simulink model "x3D_FSC_integrale"  (R2024b)
settings: Solver=FixedStepAuto  StartTime=0.0  StopTime=inf  FixedStep=0.001  RelTol=1e-3  EnableMultiTasking=on
undefined symbols (not defined in the file or in its folder): DiscIntNeverNeededParam
libraries: px4Sensorslib x5, matrix_library x4, px4Peripheralslib x1, cstblocks x1
settings Model: SimulationMode=external  ExtModeTrigDuration=10  Creator=ArriGE66  LastModifiedBy=xippa
settings SolverCC: PositivePriorityOrder=on
settings OptimizationCC: EnhancedBackFolding=on  PassReuseOutputArgsAs=Individual arguments  ZeroExternalMemoryAtStartup=off  ZeroInternalMemoryAtStartup=off  MaxStackSize=64  OptimizeBlockOrder=speed  DifferentSizesBufferReuse=on  OptimizationCustomize=off  EfficientTunableParamExpr=on
settings DebuggingCC: ParameterTunabilityLossMsg=error
settings HardwareCC: ProdBitPerPointer=32  ProdBitPerSizeT=32  ProdBitPerPtrDiffT=32  ProdLargestAtomicInteger=Long  ProdLargestAtomicFloat=Double  ProdWordSize=32  ProdLongLongMode=on  ProdHWDeviceType=ARM Compatible->ARM Cortex
settings SFSimCC: MATLABDynamicMemAlloc=off  SimTargetLang=C++
settings RTWCC: Description=Embedded Coder  SystemTargetFile=ert.tlc  HardwareBoard=PX4 Cube Orange  TemplateMakefile=ert_default_tmf  Toolchain=GNU Tools for PX4 Autopilots  TargetLang=C++  GPUComputeCapability=3.5
settings CodeAppCC: ForceParamTrailComments=on  IgnoreCustomStorageClasses=off  OperatorAnnotations=on  SimulinkDataObjDesc=on  SFDataObjDesc=on  InsertBlockDesc=on
settings ERTTargetCC: SupportVariableSizeSignals=on  ExtMode=on  ExtModeTransport=3  ExtModeStaticAlloc=on  ExtModeStaticAllocSize=1024  ExtModeMexFile=ext_xcp  ExtModeMexArgs=1 COM10 3000000  ExtModeIntrfLevel=Level2 - Open  InlinedParameterPlacement=Hierarchical  DynamicArrayContainerType=coder::array

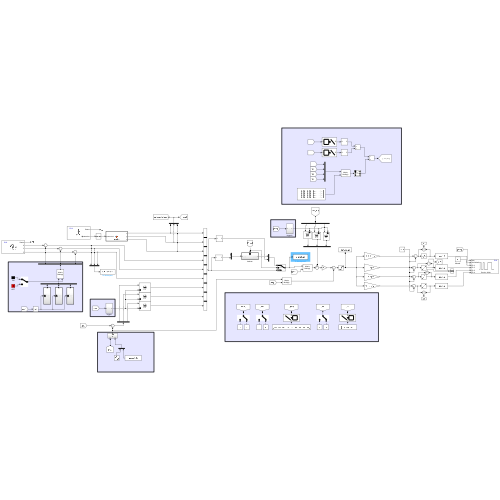
[thumbnail: Simulink's stored preview of the top-level diagram]
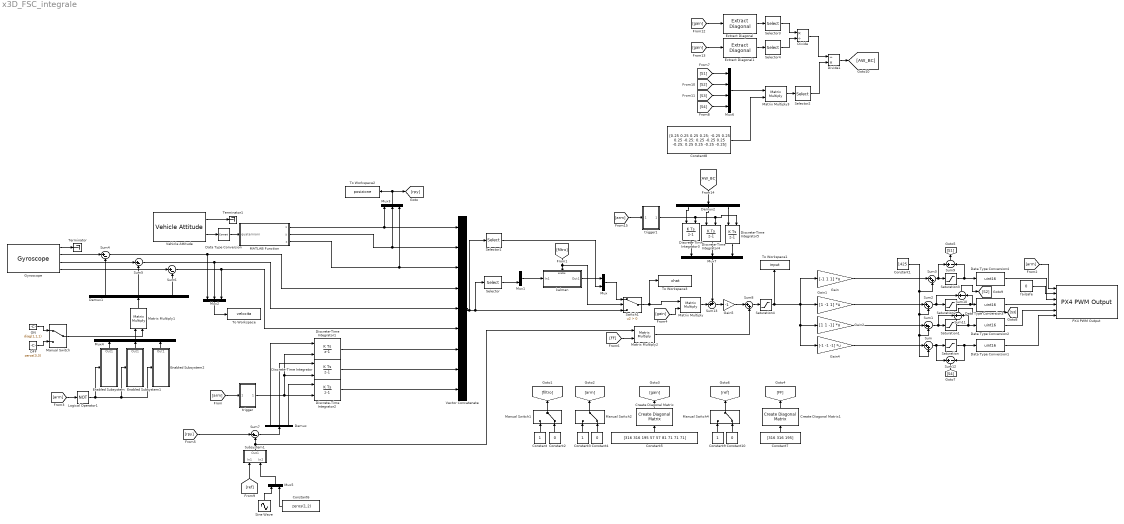
== system x3D_FSC_integrale ==
  Constant : Constant
  Constant1 : Constant  Value=1425  SampleTime=0.01
  Constant10 : Constant  Value=0
  Constant2 : Constant  Value=0
  Constant3 : Constant
  Constant4 : Constant  Value=0
  Constant5 : Constant  Value=[316 316 195 57 57 81 71 71 71]
  Constant6 : Constant  Value=zeros(1,2)
  Constant7 : Constant  Value=[316 316 195]
  Constant8 : Constant  Value=|
      | [0.25	0.25	0.25	0.25;
      | -0.25	0.25	0.25	-0.25;
      | 0.25	-0.25	0.25	-0.25;
      | 0.25	0.25	-0.25	-0.25]
  Constant9 : Constant
  Create Diagonal Matrix : matrix_library/Create Diagonal Matrix
      settings: LibrarySourceBlock=|
      | simulink/Matrix
      | Operations/Create Diagonal
      | Matrix
  Create Diagonal Matrix1 : matrix_library/Create Diagonal Matrix
      settings: LibrarySourceBlock=|
      | simulink/Matrix
      | Operations/Create Diagonal
      | Matrix
  Data Type Conversion : DataTypeConversion  SaturateOnIntegerOverflow=off  RndMeth=Floor
  Data Type Conversion{1..4} (4 alike) : DataTypeConversion  OutDataTypeStr=uint16  SaturateOnIntegerOverflow=off  RndMeth=Floor
  Demux : Demux  Outputs=3
  Demux1 : Demux  Outputs=3
  Demux2 : Demux  Outputs=3
  Discrete-Time Integrator{,1..5} (6 alike) : DiscreteIntegrator  ExternalReset=level  SampleTime=-1  ICPrevOutput=DiscIntNeverNeededParam  ICPrevScaledInput=DiscIntNeverNeededParam
  Divide : Product  Inputs=*/
  Divide1 : Product  Inputs=/*
  Enabled Subsystem : Subsystem  TreatAsAtomicUnit=on
  Enabled Subsystem1 : Subsystem  TreatAsAtomicUnit=on
  Enabled Subsystem2 : Subsystem  TreatAsAtomicUnit=on
  Extract Diagonal : matrix_library/Extract Diagonal
      settings: LibrarySourceBlock=|
      | simulink/Matrix
      | Operations/Extract Diagonal
  Extract Diagonal1 : matrix_library/Extract Diagonal
      settings: LibrarySourceBlock=|
      | simulink/Matrix
      | Operations/Extract Diagonal
  Gain : Gain  Gain=[-1 1 1]  Multiplication=Matrix(K*u)
  Gain1 : Gain  Gain=[1 -1 1]  Multiplication=Matrix(K*u)
  Gain2 : Gain  Gain=[1 1 -1]  Multiplication=Matrix(K*u)
  Gain4 : Gain  Gain=[-1 -1 -1]  Multiplication=Matrix(K*u)
  Gain5 : Gain  Gain=-1
  Gyroscope : px4Sensorslib/Gyroscope  uorbTimeStamp=off  BlockingMode=off  BlockTimeout=1e-3  sampleTime=0.01
  Logical Operator1 : Logic  Operator=NOT  AllPortsSameDT=off  OutDataTypeStr=boolean
  MATLAB Function : MATLAB Function  TreatAsAtomicUnit=on
  Manual Switch : ManualSwitch
  Manual Switch1 : ManualSwitch  CurrentSetting=0
  Manual Switch2 : ManualSwitch  CurrentSetting=0
  Manual Switch4 : ManualSwitch  CurrentSetting=0
  Matrix Multiply{,1..3} (4 alike) : Product  Multiplication=Matrix(*)
  Mux : Mux  Inputs=2
  Mux1 : Mux  Inputs=2
  Mux{2..4,7} (4 alike) : Mux  Inputs=3
  Mux5 : Mux  Inputs=2
  Mux6 : Mux
  OFF : Constant  Value=zeros(3,3)
  ON : Constant  Value=diag(1,1,1)
  PX4 PWM Output : px4Peripheralslib/PX4 PWM Output  pwmDevice=Main  pwmChannel1_=on  pwmChannel2_=on  pwmChannel3_=on  pwmChannel4_=on  pwmChannel5_=off  pwmChannel6_=off  pwmChannel7_=off  pwmChannel8_=off
  Saturation{,1..3} (4 alike) : Saturate  UpperLimit=1750  LowerLimit=1050
  Saturation4 : Saturate
  Selector : Selector  InputPortWidth=9  IndexOptions=Index vector (dialog)  Indices=[1:6]  OutputSizes=1
  Selector1 : Selector  InputPortWidth=9  IndexOptions=Index vector (dialog)  Indices=[7 8 9]  OutputSizes=1
  Selector2 : Selector  InputPortWidth=4  IndexOptions=Index vector (dialog)  Indices=[2:4]  OutputSizes=1
  Selector3 : Selector  InputPortWidth=9  IndexOptions=Index vector (dialog)  Indices=[1 2 3]  OutputSizes=1
  Selector4 : Selector  InputPortWidth=9  IndexOptions=Index vector (dialog)  Indices=[7 8 9]  OutputSizes=1
  Sine Wave : Sin  Amplitude=0.1  SampleTime=0.01
  Subsystem1 : Subsystem
  Sum{,1..3,8} (5 alike) : Sum  Inputs=|++
  Sum{9..12} (4 alike) : Sum  Inputs=+|-
  Sum13 : Sum  Inputs=++|
  Sum{4..7} (4 alike) : Sum  Inputs=|+-
  Switch1 : Switch  Criteria=u2 > Threshold  SaturateOnIntegerOverflow=off  InputSameDT=off
  Terminator : Terminator
  Terminator1 : Terminator
  To Workspace : ToWorkspace  VariableName=velocita  SaveFormat=Timeseries  SampleTime=-1
  To Workspace1 : ToWorkspace  VariableName=input  SaveFormat=Timeseries  SampleTime=-1
  To Workspace2 : ToWorkspace  VariableName=posizione  SaveFormat=Timeseries  SampleTime=-1
  To Workspace3 : ToWorkspace  VariableName=xhat  SaveFormat=Timeseries  SampleTime=-1
  Vector Concatenate : Concatenate  NumInputs=9
  Vehicle Attitude : px4Sensorslib/Vehicle Attitude  rollRate=off  pitchRate=off  yawRate=off  quaternion=on  uorbTimeStamp=off  BlockingMode=off  BlockTimeout=0.001  sampleTime=0.01
  failsafe : Constant  Value=0  OutDataTypeStr=boolean  SampleTime=0.01
  kalman : Subsystem  TreatAsAtomicUnit=on
  trigger : Subsystem
  trigger1 : Subsystem
  wires:
  Data Type Conversion2/1 -> PX4 PWM Output/5
  Data Type Conversion1/1 -> PX4 PWM Output/6
  failsafe/1 -> PX4 PWM Output/2
  Vehicle Attitude/2 -> Data Type Conversion/1
  Vehicle Attitude/1 -> Terminator1/1
  Data Type Conversion3/1 -> PX4 PWM Output/4
  Gain/1 -> Sum3/1
  Saturation3/1 -> Sum9/2, Data Type Conversion4/1
  Data Type Conversion4/1 -> PX4 PWM Output/3
  Sum3/1 -> Sum9/1, Saturation3/1
  Constant1/1 -> Sum/2, Sum1/2, Sum2/2, Sum3/2
  Vector Concatenate/1 -> Selector1/1, Selector/1, Switch1/3
  Gain1/1 -> Sum2/1
  Gain2/1 -> Sum1/1
  Gain4/1 -> Sum/1
  Selector/1 -> Mux1/2
  [filtro] -> Switch1/2, kalman/Enable
  kalman/1(Out1) -> Mux/1
  Selector1/1 -> Mux/2
  Mux/1 -> Switch1/1
  Mux1/1 -> kalman/1(In1)
  Data Type Conversion/1 -> MATLAB Function/1(quaternioni)
  Switch1/1 -> To Workspace3/1, Matrix Multiply/1
  trigger/1(Out1) -> Discrete-Time Integrator1/2, Discrete-Time Integrator/2, Discrete-Time Integrator2/2
  [arm] -> trigger/1(In1)
  Sum4/1 -> Vector Concatenate/4, Mux2/1
  ON/1 -> Manual Switch/1
  Gyroscope/4 -> Sum6/1
  Manual Switch/1 -> Matrix Multiply1/2
  Demux1/2 -> Sum5/2
  Matrix Multiply1/1 -> Demux1/1
  Gyroscope/2 -> Sum4/1
  Gyroscope/3 -> Sum5/1
  OFF/1 -> Manual Switch/2
  Sum5/1 -> Vector Concatenate/5, Mux2/2
  Demux1/3 -> Sum6/2
  Demux1/1 -> Sum4/2
  Gyroscope/1 -> Terminator/1
  Sum6/1 -> Mux2/3, Vector Concatenate/6
  Logical Operator1/1 -> Enabled Subsystem2/Enable, Enabled Subsystem1/Enable, Enabled Subsystem/Enable
  Enabled Subsystem2/1(Out1) -> Mux4/3
  Enabled Subsystem/1(Out1) -> Mux4/1
  [arm] -> Logical Operator1/1
  Enabled Subsystem1/1(Out1) -> Mux4/2
  Mux4/1 -> Matrix Multiply1/1
  Manual Switch1/1 -> [filtro]
  Constant2/1 -> Manual Switch1/2
  Constant/1 -> Manual Switch1/1
  [arm] -> PX4 PWM Output/1
  Constant3/1 -> Manual Switch2/1
  Manual Switch2/1 -> [arm]
  Constant4/1 -> Manual Switch2/2
  [gain] -> Matrix Multiply/2
  Create Diagonal Matrix/1 -> [gain]
  Constant5/1 -> Create Diagonal Matrix/1
  Mux2/1 -> To Workspace/1
  MATLAB Function/1(x) -> Mux3/1, Vector Concatenate/1
  MATLAB Function/2(y) -> Mux3/2, Vector Concatenate/2
  MATLAB Function/3(z) -> Mux3/3, Vector Concatenate/3
  Discrete-Time Integrator1/1 -> Vector Concatenate/7
  Discrete-Time Integrator/1 -> Vector Concatenate/8
  Discrete-Time Integrator2/1 -> Vector Concatenate/9
  Mux3/1 -> [rpy], To Workspace2/1
  Manual Switch4/1 -> [ref]
  Constant9/1 -> Manual Switch4/1
  Constant10/1 -> Manual Switch4/2
  [ref] -> Subsystem1/1(In1)
  Sine Wave/1 -> Mux5/1
  Mux5/1 -> Subsystem1/2(In2)
  Constant6/1 -> Mux5/2
  [rpy] -> Sum7/1
  Sum7/1 -> Demux/1
  Demux/1 -> Discrete-Time Integrator1/1
  Demux/2 -> Discrete-Time Integrator/1
  Demux/3 -> Discrete-Time Integrator2/1
  Gain5/1 -> Sum8/1
  Sum8/1 -> Saturation4/1
  Matrix Multiply2/1 -> Sum8/2
  Subsystem1/1(Out1) -> Matrix Multiply2/1, Sum7/2
  [FF] -> Matrix Multiply2/2
  Create Diagonal Matrix1/1 -> [FF]
  Constant7/1 -> Create Diagonal Matrix1/1
  Saturation4/1 -> Gain4/1, Gain2/1, Gain1/1, Gain/1, To Workspace1/1
  Saturation2/1 -> Sum10/2, Data Type Conversion3/1
  Sum2/1 -> Sum10/1, Saturation2/1
  Saturation1/1 -> Sum11/2, Data Type Conversion2/1
  Sum1/1 -> Sum11/1, Saturation1/1
  Saturation/1 -> Sum12/2, Data Type Conversion1/1
  Sum/1 -> Sum12/1, Saturation/1
  Sum9/1 -> [S1]
  Sum12/1 -> [S4]
  Sum11/1 -> [S3]
  Sum10/1 -> [S2]
  [S2] -> Mux6/2
  [S1] -> Mux6/1
  [S3] -> Mux6/3
  [S4] -> Mux6/4
  Mux6/1 -> Matrix Multiply3/1
  Constant8/1 -> Matrix Multiply3/2
  Matrix Multiply3/1 -> Selector2/1
  [gain] -> Extract Diagonal/1
  Extract Diagonal/1 -> Selector3/1
  [gain] -> Extract Diagonal1/1
  Extract Diagonal1/1 -> Selector4/1
  Selector3/1 -> Divide/1
  Selector4/1 -> Divide/2
  Divide/1 -> Divide1/1
  Selector2/1 -> Divide1/2
  Divide1/1 -> [AW_BC]
  Matrix Multiply/1 -> Sum13/2
  [AW_BC] -> Demux2/1
  [arm] -> trigger1/1(In1)
  Demux2/3 -> Discrete-Time Integrator5/1
  Demux2/2 -> Discrete-Time Integrator4/1
  Demux2/1 -> Discrete-Time Integrator3/1
  trigger1/1(Out1) -> Discrete-Time Integrator5/2, Discrete-Time Integrator4/2, Discrete-Time Integrator3/2
  Sum13/1 -> Gain5/1
  Discrete-Time Integrator3/1 -> Mux7/1
  Discrete-Time Integrator5/1 -> Mux7/3
  Discrete-Time Integrator4/1 -> Mux7/2
  Mux7/1 -> Sum13/1

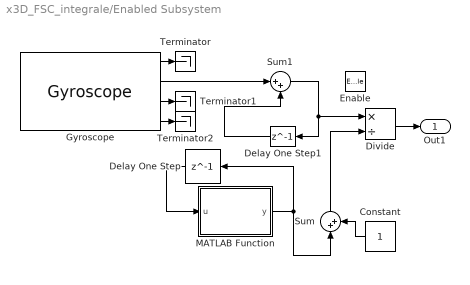
== system x3D_FSC_integrale/Enabled Subsystem ==
  Enable : EnablePort
  Constant : Constant
  Delay One Step : Delay  DelayLength=1
  Delay One Step1 : Delay  DelayLength=1
  Divide : Product  Inputs=*/
  Gyroscope : px4Sensorslib/Gyroscope  uorbTimeStamp=off  BlockingMode=off  BlockTimeout=1e-3  sampleTime=0.01
  MATLAB Function : MATLAB Function  TreatAsAtomicUnit=on
  Sum : Sum  Inputs=|++
  Sum1 : Sum  Inputs=|++
  Terminator : Terminator
  Terminator1 : Terminator
  Terminator2 : Terminator
  Out1 : Outport
  wires:
  Divide/1 -> Out1/1
  Sum1/1 -> Delay One Step1/1, Divide/1
  Sum/1 -> Divide/2
  Constant/1 -> Sum/2
  MATLAB Function/1(y) -> Delay One Step/1, Sum/1
  Delay One Step/1 -> MATLAB Function/1(u)
  Delay One Step1/1 -> Sum1/2
  Gyroscope/4 -> Terminator2/1
  Gyroscope/3 -> Terminator1/1
  Gyroscope/1 -> Terminator/1
  Gyroscope/2 -> Sum1/1

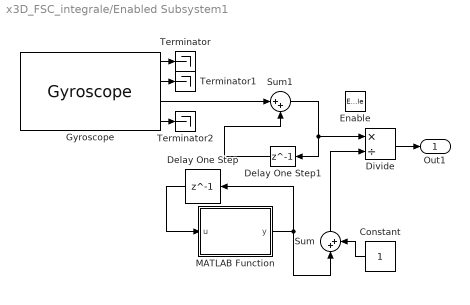
== system x3D_FSC_integrale/Enabled Subsystem1 ==
  Enable : EnablePort
  Constant : Constant
  Delay One Step : Delay  DelayLength=1
  Delay One Step1 : Delay  DelayLength=1
  Divide : Product  Inputs=*/
  Gyroscope : px4Sensorslib/Gyroscope  uorbTimeStamp=off  BlockingMode=off  BlockTimeout=1e-3  sampleTime=0.01
  MATLAB Function : MATLAB Function  TreatAsAtomicUnit=on
  Sum : Sum  Inputs=|++
  Sum1 : Sum  Inputs=|++
  Terminator : Terminator
  Terminator1 : Terminator
  Terminator2 : Terminator
  Out1 : Outport
  wires:
  Divide/1 -> Out1/1
  Sum1/1 -> Delay One Step1/1, Divide/1
  Sum/1 -> Divide/2
  Constant/1 -> Sum/2
  MATLAB Function/1(y) -> Delay One Step/1, Sum/1
  Delay One Step/1 -> MATLAB Function/1(u)
  Delay One Step1/1 -> Sum1/2
  Gyroscope/4 -> Terminator2/1
  Gyroscope/1 -> Terminator/1
  Gyroscope/3 -> Sum1/1
  Gyroscope/2 -> Terminator1/1

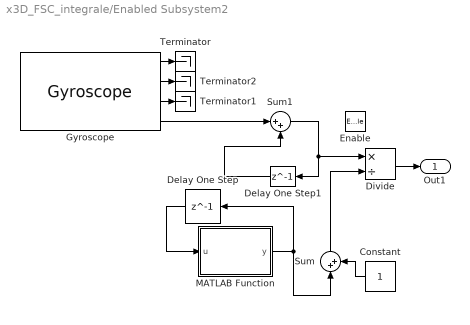
== system x3D_FSC_integrale/Enabled Subsystem2 ==
  Enable : EnablePort
  Constant : Constant
  Delay One Step : Delay  DelayLength=1
  Delay One Step1 : Delay  DelayLength=1
  Divide : Product  Inputs=*/
  Gyroscope : px4Sensorslib/Gyroscope  uorbTimeStamp=off  BlockingMode=off  BlockTimeout=1e-3  sampleTime=0.01
  MATLAB Function : MATLAB Function  TreatAsAtomicUnit=on
  Sum : Sum  Inputs=|++
  Sum1 : Sum  Inputs=|++
  Terminator : Terminator
  Terminator1 : Terminator
  Terminator2 : Terminator
  Out1 : Outport
  wires:
  Divide/1 -> Out1/1
  Sum1/1 -> Delay One Step1/1, Divide/1
  Sum/1 -> Divide/2
  Constant/1 -> Sum/2
  MATLAB Function/1(y) -> Delay One Step/1, Sum/1
  Delay One Step/1 -> MATLAB Function/1(u)
  Delay One Step1/1 -> Sum1/2
  Gyroscope/3 -> Terminator1/1
  Gyroscope/1 -> Terminator/1
  Gyroscope/4 -> Sum1/1
  Gyroscope/2 -> Terminator2/1

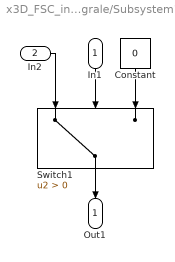
== system x3D_FSC_integrale/Subsystem1 ==
  In1 : Inport
  In2 : Inport  Port=2
  Constant : Constant  Value=0
  Switch1 : Switch  Criteria=u2 > Threshold  SaturateOnIntegerOverflow=off  InputSameDT=off
  Out1 : Outport
  wires:
  Switch1/1 -> Out1/1
  In1/1 -> Switch1/2
  Constant/1 -> Switch1/3
  In2/1 -> Switch1/1

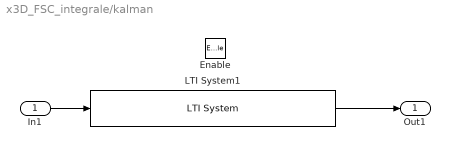
== system x3D_FSC_integrale/kalman ==
  In1 : Inport
  Enable : EnablePort
  LTI System1 : cstblocks/LTI System  sys=kalmand  IC=[0 0 0 0 0 0]  PadeOrder=0
  Out1 : Outport
  wires:
  In1/1 -> LTI System1/1
  LTI System1/1 -> Out1/1

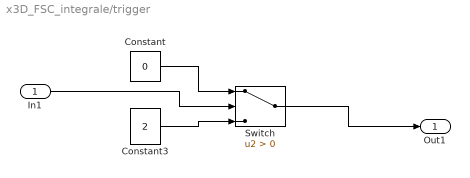
== system x3D_FSC_integrale/trigger ==
  In1 : Inport
  Constant : Constant  Value=0
  Constant3 : Constant  Value=2
  Switch : Switch  Criteria=u2 > Threshold  SaturateOnIntegerOverflow=off  InputSameDT=off
  Out1 : Outport
  wires:
  Constant/1 -> Switch/1
  Constant3/1 -> Switch/3
  Switch/1 -> Out1/1
  In1/1 -> Switch/2

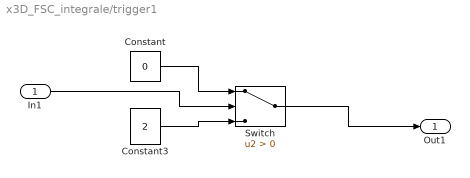
== system x3D_FSC_integrale/trigger1 ==
  In1 : Inport
  Constant : Constant  Value=0
  Constant3 : Constant  Value=2
  Switch : Switch  Criteria=u2 > Threshold  SaturateOnIntegerOverflow=off  InputSameDT=off
  Out1 : Outport
  wires:
  Constant/1 -> Switch/1
  Constant3/1 -> Switch/3
  Switch/1 -> Out1/1
  In1/1 -> Switch/2

== matlab function x3D_FSC_integrale/Enabled Subsystem/MATLAB Function ==
  data: u input; y output
function y = fcn(u)
y = u+1;

== matlab function x3D_FSC_integrale/Enabled Subsystem1/MATLAB Function ==
  data: u input; y output
function y = fcn(u)
y = u+1;

== matlab function x3D_FSC_integrale/Enabled Subsystem2/MATLAB Function ==
  data: u input; y output
function y = fcn(u)
y = u+1;

== matlab function x3D_FSC_integrale/MATLAB Function ==
  data: x output; y output; quaternioni input; z output
function [x, y, z] = assetto(quaternioni)
    % Estrazione dei componenti del quaternione
    qw = quaternioni(1);
    qx = quaternioni(2);
    qy = quaternioni(3);
    qz = quaternioni(4);

    % Calcolo degli angoli di Eulero manualmente
    x = atan2(2*(qw*qx + qy*qz), 1 - 2*(qx^2 + qy^2)); % roll
    y = asin(2*(qw*qy - qz*qx));                          % Pitch
    z = atan2(2*(qw*qz + qx*qy), 1 - 2*(qy^2 + qz^2));   % yaw
end
